simulink model "flappy_hk_disturbed_position_hover"  (R2024a)
settings: Solver=ode15s  StartTime=0.0  StopTime=5  MaxStep=0.0001  RelTol=1e-3
undefined symbols (not defined in the file): flappy_sil_position_controller, flappy_sil_sensor_model, flappy_sil_virtual_actuator, flappy_sil_wing_kinematics, flappy_sil_wing_loads, X, Y, Z
libraries: sm_lib x66, nesl_utility x36
(part 1 of 2)
settings Model: Creator=10049  LastModifiedBy=10049
settings DataIOCC: SaveFormat=StructureWithTime

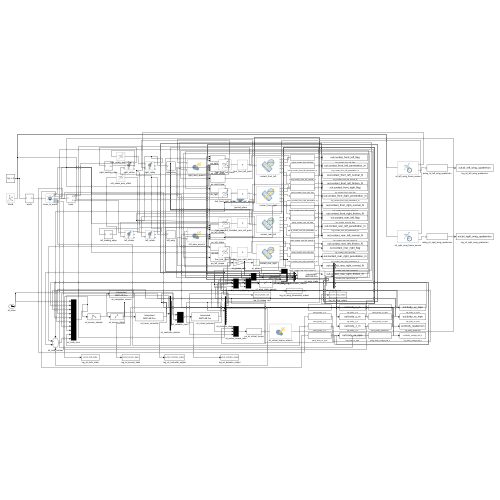
[thumbnail: Simulink's stored preview of the top-level diagram]
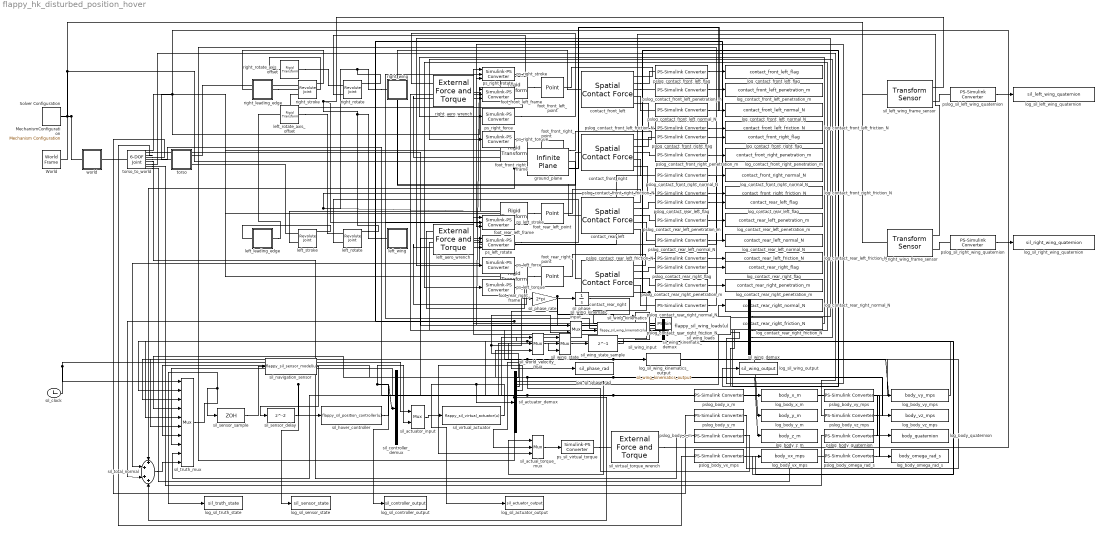
== system flappy_hk_disturbed_position_hover ==
  MechanismConfiguration : sm_lib/Utilities/Mechanism Configuration  UniformGravity=Constant  GravityVector=[0 0 -9.80665]  GravityVectorUnits=m/s^2  LinearizationDelta=0.001  JointModeTransitionNonlinearIterations=2
  Solver Configuration : nesl_utility/Solver Configuration  PhysicalDomain=network_engine_domain  SubClassName=solver  LeftPortType=input  RightPortType=generic  Tones=[]  Harmonics=[]  SimulateNoise=off  Profile=off  UseLocalSampling=off  EnableSwitchedLinearOptims=on  FrequencyDomain=off  UseCCode=off  RelTol=0.001  AbsTol=0.001  MinStep=1e-09  ToWorkspace=off  RevertToSquareIcSolve=off  NumHomotopyIterations=100  PhasorMode=off  PhasorModeNumHarmonics=1  ConsistencySolver=NEWTON_XTOL_AFTER_FTOL  IndexReductionMethod=DerivativeReplacement  DoDC=off  ResidualTolerance=1e-09  ConsistencyTolSource=GLOBAL  ConsistencyAbsTol=0.001  ConsistencyRelTol=0.001  ConsistencyTolFactor=0.001  UseLocalSolver=off  LocalSolverChoice=NE_BACKWARD_EULER_ADVANCER  ResolveIndetEquations=on  FunctionEvalNumThread=1  LocalSolverSampleTime=0.001  DoFixedCost=off  MaxNonlinIter=3  MaxModeIter=2  ComputeImpulses=off  ImpulseIterations=2  LinearAlgebra=auto  LinearAlgebraNumThread=0  EquationFormulation=NE_TIME_EF  DelaysMemoryBudget=1024  AutomaticFiltering=on  FilteringTimeConstant=0.001  PartitionStorageMethod=AS_NEEDED  PartitionMemoryBudget=1024  PartitionMethod=ROBUST  MultibodyUseLocalSolver=off  MultibodyLocalSolverChoice=ODE1  MultibodyLocalSolverSampleTime=0.001
  World : sm_lib/Frames and Transforms/World Frame
  contact_front_left : sm_lib/Forces and Torques/Spatial Contact Force  NormalForceType=SmoothSpringDamper  NormalStiffness=996.3556  NormalStiffnessUnits=N/m  NormalDamping=9.9602  NormalDampingUnits=N/(m/s)  NormalTransitionRegionWidth=0.0001  NormalTransitionRegionWidthUnits=m  FrictionType=SmoothStickSlip  CoefficientOfStaticFriction=0.6  CoefficientOfDynamicFriction=0.5  FrictionalCriticalVelocity=0.01  FrictionalCriticalVelocityUnits=m/s  SenseContactSignal=on  SensePenetrationDepth=on  SenseSeparationDistance=off  SenseNormalForceMagnitude=on  SenseFrictionalForceMagnitude=on  SenseNormalVelocity=off  SenseTangentialVelocity=off  SenseContactBaseRotation=off  SenseContactBaseTranslation=off  SenseContactFollowerRotation=off  SenseContactFollowerTranslation=off  ZeroCrossDetectContactStartAndEnd=on
  contact_front_right : sm_lib/Forces and Torques/Spatial Contact Force  NormalForceType=SmoothSpringDamper  NormalStiffness=996.3556  NormalStiffnessUnits=N/m  NormalDamping=9.9602  NormalDampingUnits=N/(m/s)  NormalTransitionRegionWidth=0.0001  NormalTransitionRegionWidthUnits=m  FrictionType=SmoothStickSlip  CoefficientOfStaticFriction=0.6  CoefficientOfDynamicFriction=0.5  FrictionalCriticalVelocity=0.01  FrictionalCriticalVelocityUnits=m/s  SenseContactSignal=on  SensePenetrationDepth=on  SenseSeparationDistance=off  SenseNormalForceMagnitude=on  SenseFrictionalForceMagnitude=on  SenseNormalVelocity=off  SenseTangentialVelocity=off  SenseContactBaseRotation=off  SenseContactBaseTranslation=off  SenseContactFollowerRotation=off  SenseContactFollowerTranslation=off  ZeroCrossDetectContactStartAndEnd=on
  contact_rear_left : sm_lib/Forces and Torques/Spatial Contact Force  NormalForceType=SmoothSpringDamper  NormalStiffness=996.3556  NormalStiffnessUnits=N/m  NormalDamping=9.9602  NormalDampingUnits=N/(m/s)  NormalTransitionRegionWidth=0.0001  NormalTransitionRegionWidthUnits=m  FrictionType=SmoothStickSlip  CoefficientOfStaticFriction=0.6  CoefficientOfDynamicFriction=0.5  FrictionalCriticalVelocity=0.01  FrictionalCriticalVelocityUnits=m/s  SenseContactSignal=on  SensePenetrationDepth=on  SenseSeparationDistance=off  SenseNormalForceMagnitude=on  SenseFrictionalForceMagnitude=on  SenseNormalVelocity=off  SenseTangentialVelocity=off  SenseContactBaseRotation=off  SenseContactBaseTranslation=off  SenseContactFollowerRotation=off  SenseContactFollowerTranslation=off  ZeroCrossDetectContactStartAndEnd=on
  contact_rear_right : sm_lib/Forces and Torques/Spatial Contact Force  NormalForceType=SmoothSpringDamper  NormalStiffness=996.3556  NormalStiffnessUnits=N/m  NormalDamping=9.9602  NormalDampingUnits=N/(m/s)  NormalTransitionRegionWidth=0.0001  NormalTransitionRegionWidthUnits=m  FrictionType=SmoothStickSlip  CoefficientOfStaticFriction=0.6  CoefficientOfDynamicFriction=0.5  FrictionalCriticalVelocity=0.01  FrictionalCriticalVelocityUnits=m/s  SenseContactSignal=on  SensePenetrationDepth=on  SenseSeparationDistance=off  SenseNormalForceMagnitude=on  SenseFrictionalForceMagnitude=on  SenseNormalVelocity=off  SenseTangentialVelocity=off  SenseContactBaseRotation=off  SenseContactBaseTranslation=off  SenseContactFollowerRotation=off  SenseContactFollowerTranslation=off  ZeroCrossDetectContactStartAndEnd=on
  foot_front_left_frame : sm_lib/Frames and Transforms/Rigid Transform  RotationMethod=None  FollAlignAxisA=+X  BaseAlignAxisA=+Y  FollAlignAxisB=+Y  BaseAlignAxisB=+Z  RotationStandardAxis=+Z  RotationAngle=0  RotationAngleUnits=deg  RotationArbitraryAxis=[0 0 1]  RotationSequenceAxes=FollowerAxes  RotationSequence=XYX  RotationSequenceAngles=[0 0 0]  RotationSequenceAnglesUnits=deg  RotationMatrix=[1 0 0;0 1 0;0 0 1]  Quaternion=[1 0 0 0]  TranslationMethod=Cartesian  TranslationCartesianOffset=[-0.056123561 -0.056123561 -0.0610087]  TranslationCartesianOffsetUnits=m  TranslationStandardAxis=+Z  TranslationStandardOffset=0  TranslationStandardOffsetUnits=m  TranslationROffset=0  TranslationROffsetUnits=m  TranslationThetaOffset=0  TranslationThetaOffsetUnits=deg  TranslationZOffset=0  TranslationZOffsetUnits=m
  foot_front_left_point : sm_lib/Curves and Surfaces/Point  GraphicType=Marker  MarkerShape=Sphere  MarkerSize=10  GraphicVisPropType=SimpleVisualProperties  GraphicDiffuseColor=[0.5 0.5 0.5]  GraphicOpacity=1  GraphicSpecularColor=[0.5 0.5 0.5 1.0]  GraphicAmbientColor=[0.15 0.15 0.15 1.0]  GraphicEmissiveColor=[0.0 0.0 0.0 1.0]  GraphicShininess=75
  foot_front_right_frame : sm_lib/Frames and Transforms/Rigid Transform  RotationMethod=None  FollAlignAxisA=+X  BaseAlignAxisA=+Y  FollAlignAxisB=+Y  BaseAlignAxisB=+Z  RotationStandardAxis=+Z  RotationAngle=0  RotationAngleUnits=deg  RotationArbitraryAxis=[0 0 1]  RotationSequenceAxes=FollowerAxes  RotationSequence=XYX  RotationSequenceAngles=[0 0 0]  RotationSequenceAnglesUnits=deg  RotationMatrix=[1 0 0;0 1 0;0 0 1]  Quaternion=[1 0 0 0]  TranslationMethod=Cartesian  TranslationCartesianOffset=[-0.056123561 0.056123557 -0.0610087]  TranslationCartesianOffsetUnits=m  TranslationStandardAxis=+Z  TranslationStandardOffset=0  TranslationStandardOffsetUnits=m  TranslationROffset=0  TranslationROffsetUnits=m  TranslationThetaOffset=0  TranslationThetaOffsetUnits=deg  TranslationZOffset=0  TranslationZOffsetUnits=m
  foot_front_right_point : sm_lib/Curves and Surfaces/Point  GraphicType=Marker  MarkerShape=Sphere  MarkerSize=10  GraphicVisPropType=SimpleVisualProperties  GraphicDiffuseColor=[0.5 0.5 0.5]  GraphicOpacity=1  GraphicSpecularColor=[0.5 0.5 0.5 1.0]  GraphicAmbientColor=[0.15 0.15 0.15 1.0]  GraphicEmissiveColor=[0.0 0.0 0.0 1.0]  GraphicShininess=75
  foot_rear_left_frame : sm_lib/Frames and Transforms/Rigid Transform  RotationMethod=None  FollAlignAxisA=+X  BaseAlignAxisA=+Y  FollAlignAxisB=+Y  BaseAlignAxisB=+Z  RotationStandardAxis=+Z  RotationAngle=0  RotationAngleUnits=deg  RotationArbitraryAxis=[0 0 1]  RotationSequenceAxes=FollowerAxes  RotationSequence=XYX  RotationSequenceAngles=[0 0 0]  RotationSequenceAnglesUnits=deg  RotationMatrix=[1 0 0;0 1 0;0 0 1]  Quaternion=[1 0 0 0]  TranslationMethod=Cartesian  TranslationCartesianOffset=[0.056357642 -0.056357654 -0.0610087]  TranslationCartesianOffsetUnits=m  TranslationStandardAxis=+Z  TranslationStandardOffset=0  TranslationStandardOffsetUnits=m  TranslationROffset=0  TranslationROffsetUnits=m  TranslationThetaOffset=0  TranslationThetaOffsetUnits=deg  TranslationZOffset=0  TranslationZOffsetUnits=m
  foot_rear_left_point : sm_lib/Curves and Surfaces/Point  GraphicType=Marker  MarkerShape=Sphere  MarkerSize=10  GraphicVisPropType=SimpleVisualProperties  GraphicDiffuseColor=[0.5 0.5 0.5]  GraphicOpacity=1  GraphicSpecularColor=[0.5 0.5 0.5 1.0]  GraphicAmbientColor=[0.15 0.15 0.15 1.0]  GraphicEmissiveColor=[0.0 0.0 0.0 1.0]  GraphicShininess=75
  foot_rear_right_frame : sm_lib/Frames and Transforms/Rigid Transform  RotationMethod=None  FollAlignAxisA=+X  BaseAlignAxisA=+Y  FollAlignAxisB=+Y  BaseAlignAxisB=+Z  RotationStandardAxis=+Z  RotationAngle=0  RotationAngleUnits=deg  RotationArbitraryAxis=[0 0 1]  RotationSequenceAxes=FollowerAxes  RotationSequence=XYX  RotationSequenceAngles=[0 0 0]  RotationSequenceAnglesUnits=deg  RotationMatrix=[1 0 0;0 1 0;0 0 1]  Quaternion=[1 0 0 0]  TranslationMethod=Cartesian  TranslationCartesianOffset=[0.056357642 0.056357642 -0.0610087]  TranslationCartesianOffsetUnits=m  TranslationStandardAxis=+Z  TranslationStandardOffset=0  TranslationStandardOffsetUnits=m  TranslationROffset=0  TranslationROffsetUnits=m  TranslationThetaOffset=0  TranslationThetaOffsetUnits=deg  TranslationZOffset=0  TranslationZOffsetUnits=m
  foot_rear_right_point : sm_lib/Curves and Surfaces/Point  GraphicType=Marker  MarkerShape=Sphere  MarkerSize=10  GraphicVisPropType=SimpleVisualProperties  GraphicDiffuseColor=[0.5 0.5 0.5]  GraphicOpacity=1  GraphicSpecularColor=[0.5 0.5 0.5 1.0]  GraphicAmbientColor=[0.15 0.15 0.15 1.0]  GraphicEmissiveColor=[0.0 0.0 0.0 1.0]  GraphicShininess=75
  ground_plane : sm_lib/Curves and Surfaces/Infinite Plane  GraphicType=Rectangle  GraphicPlaneWidth=3  GraphicPlaneWidthUnits=m  GraphicPlaneHeight=3  GraphicPlaneHeightUnits=m  GraphicVisPropType=SimpleVisualProperties  GraphicDiffuseColor=[0.93 0.94 0.96]  GraphicOpacity=0.98  GraphicSpecularColor=[0.06 0.06 0.07 1]  GraphicAmbientColor=[0.2 0.2 0.2 1]  GraphicEmissiveColor=[0 0 0 1]  GraphicShininess=4
  left_aero_wrench : sm_lib/Forces and Torques/External Force and Torque  EnableForceX=off  EnableForceY=off  EnableForceZ=off  EnableForce=on  ForceResolutionFrame=World  EnableTorqueX=off  EnableTorqueY=off  EnableTorqueZ=off  EnableTorque=on  TorqueResolutionFrame=World
  left_leading_edge : Subsystem
  left_rotate : sm_lib/Joints/Revolute Joint  JointMode=Normal  CompositeWrenchDir=FollowerOnBase  CompositeWrenchFrame=BaseFrame  SenseConstraintForce=off  SenseConstraintTorque=off  SenseTotalForce=off  SenseTotalTorque=off  PositionTargetSpecify=off  PositionTargetPriority=High  PositionTargetValue=0  PositionTargetValueUnits=deg  VelocityTargetSpecify=off  VelocityTargetPriority=High  VelocityTargetValue=0  VelocityTargetValueUnits=deg/s  EquilibriumPosition=0  EquilibriumPositionUnits=deg  SpringStiffness=0  SpringStiffnessUnits=N*m/deg  DampingCoefficient=1e-9  DampingCoefficientUnits=kg*m^2/(rad*s)  LowerLimitSpecify=on  LowerLimitBound=-0.7854  LowerLimitBoundUnits=rad  LowerLimitStiffness=1e4  LowerLimitStiffnessUnits=N*m/deg  LowerLimitDamping=10  LowerLimitDampingUnits=N*m/(deg/s)  LowerLimitTransitionRegionWidth=0.1  LowerLimitTransitionRegionWidthUnits=deg  UpperLimitSpecify=on  UpperLimitBound=0.7854  UpperLimitBoundUnits=rad  UpperLimitStiffness=1e4  UpperLimitStiffnessUnits=N*m/deg  UpperLimitDamping=10  UpperLimitDampingUnits=N*m/(deg/s)  UpperLimitTransitionRegionWidth=0.1  UpperLimitTransitionRegionWidthUnits=deg  TorqueActuationMode=ComputedTorque  MotionActuationMode=InputMotion  SensePosition=on  SenseVelocity=on  SenseAcceleration=off  SenseTorqueForce=off  SenseLowerLimitTorqueForce=off  SenseUpperLimitTorqueForce=off
  left_rotate_axis_offset : sm_lib/Frames and Transforms/Rigid Transform  RotationMethod=None  FollAlignAxisA=+X  BaseAlignAxisA=+Y  FollAlignAxisB=+Y  BaseAlignAxisB=+Z  RotationStandardAxis=+Z  RotationAngle=0  RotationAngleUnits=deg  RotationArbitraryAxis=[0 0 1]  RotationSequenceAxes=FollowerAxes  RotationSequence=XYX  RotationSequenceAngles=[0 0 0]  RotationSequenceAnglesUnits=deg  RotationMatrix=[1 0 0;0 1 0;0 0 1]  Quaternion=[1 0 0 0]  TranslationMethod=Cartesian  TranslationCartesianOffset=[0 0 0]  TranslationCartesianOffsetUnits=m  TranslationStandardAxis=+Z  TranslationStandardOffset=0  TranslationStandardOffsetUnits=m  TranslationROffset=0  TranslationROffsetUnits=m  TranslationThetaOffset=0  TranslationThetaOffsetUnits=deg  TranslationZOffset=0  TranslationZOffsetUnits=m
  left_stroke : sm_lib/Joints/Revolute Joint  JointMode=Normal  CompositeWrenchDir=FollowerOnBase  CompositeWrenchFrame=BaseFrame  SenseConstraintForce=off  SenseConstraintTorque=off  SenseTotalForce=off  SenseTotalTorque=off  PositionTargetSpecify=off  PositionTargetPriority=High  PositionTargetValue=0  PositionTargetValueUnits=deg  VelocityTargetSpecify=off  VelocityTargetPriority=High  VelocityTargetValue=0  VelocityTargetValueUnits=deg/s  EquilibriumPosition=0  EquilibriumPositionUnits=deg  SpringStiffness=0.013384  SpringStiffnessUnits=N*m/deg  DampingCoefficient=8e-9  DampingCoefficientUnits=kg*m^2/(rad*s)  LowerLimitSpecify=on  LowerLimitBound=-1.63  LowerLimitBoundUnits=rad  LowerLimitStiffness=1e4  LowerLimitStiffnessUnits=N*m/deg  LowerLimitDamping=10  LowerLimitDampingUnits=N*m/(deg/s)  LowerLimitTransitionRegionWidth=0.1  LowerLimitTransitionRegionWidthUnits=deg  UpperLimitSpecify=on  UpperLimitBound=1.63  UpperLimitBoundUnits=rad  UpperLimitStiffness=1e4  UpperLimitStiffnessUnits=N*m/deg  UpperLimitDamping=10  UpperLimitDampingUnits=N*m/(deg/s)  UpperLimitTransitionRegionWidth=0.1  UpperLimitTransitionRegionWidthUnits=deg  TorqueActuationMode=ComputedTorque  MotionActuationMode=InputMotion  SensePosition=on  SenseVelocity=on  SenseAcceleration=off  SenseTorqueForce=off  SenseLowerLimitTorqueForce=off  SenseUpperLimitTorqueForce=off
  left_wing : Subsystem
  log_body_omega_rad_s : ToWorkspace  VariableName=body_omega_rad_s  SaveFormat=Structure With Time  SampleTime=-1
  log_body_quaternion : ToWorkspace  VariableName=body_quaternion  SaveFormat=Structure With Time  SampleTime=-1
  log_body_vx_mps : ToWorkspace  VariableName=body_vx_mps  SaveFormat=Structure With Time  SampleTime=-1
  log_body_vy_mps : ToWorkspace  VariableName=body_vy_mps  SaveFormat=Structure With Time  SampleTime=-1
  log_body_vz_mps : ToWorkspace  VariableName=body_vz_mps  SaveFormat=Structure With Time  SampleTime=-1
  log_body_x_m : ToWorkspace  VariableName=body_x_m  SaveFormat=Structure With Time  SampleTime=-1
  log_body_y_m : ToWorkspace  VariableName=body_y_m  SaveFormat=Structure With Time  SampleTime=-1
  log_body_z_m : ToWorkspace  VariableName=body_z_m  SaveFormat=Structure With Time  SampleTime=-1
  log_contact_front_left_flag : ToWorkspace  VariableName=contact_front_left_flag  SaveFormat=Structure With Time  SampleTime=-1
  log_contact_front_left_friction_N : ToWorkspace  VariableName=contact_front_left_friction_N  SaveFormat=Structure With Time  SampleTime=-1
  log_contact_front_left_normal_N : ToWorkspace  VariableName=contact_front_left_normal_N  SaveFormat=Structure With Time  SampleTime=-1
  log_contact_front_left_penetration_m : ToWorkspace  VariableName=contact_front_left_penetration_m  SaveFormat=Structure With Time  SampleTime=-1
  log_contact_front_right_flag : ToWorkspace  VariableName=contact_front_right_flag  SaveFormat=Structure With Time  SampleTime=-1
  log_contact_front_right_friction_N : ToWorkspace  VariableName=contact_front_right_friction_N  SaveFormat=Structure With Time  SampleTime=-1
  log_contact_front_right_normal_N : ToWorkspace  VariableName=contact_front_right_normal_N  SaveFormat=Structure With Time  SampleTime=-1
  log_contact_front_right_penetration_m : ToWorkspace  VariableName=contact_front_right_penetration_m  SaveFormat=Structure With Time  SampleTime=-1
  log_contact_rear_left_flag : ToWorkspace  VariableName=contact_rear_left_flag  SaveFormat=Structure With Time  SampleTime=-1
  log_contact_rear_left_friction_N : ToWorkspace  VariableName=contact_rear_left_friction_N  SaveFormat=Structure With Time  SampleTime=-1
  log_contact_rear_left_normal_N : ToWorkspace  VariableName=contact_rear_left_normal_N  SaveFormat=Structure With Time  SampleTime=-1
  log_contact_rear_left_penetration_m : ToWorkspace  VariableName=contact_rear_left_penetration_m  SaveFormat=Structure With Time  SampleTime=-1
  log_contact_rear_right_flag : ToWorkspace  VariableName=contact_rear_right_flag  SaveFormat=Structure With Time  SampleTime=-1
  log_contact_rear_right_friction_N : ToWorkspace  VariableName=contact_rear_right_friction_N  SaveFormat=Structure With Time  SampleTime=-1
  log_contact_rear_right_normal_N : ToWorkspace  VariableName=contact_rear_right_normal_N  SaveFormat=Structure With Time  SampleTime=-1
  log_contact_rear_right_penetration_m : ToWorkspace  VariableName=contact_rear_right_penetration_m  SaveFormat=Structure With Time  SampleTime=-1
  log_sil_actuator_output : ToWorkspace  VariableName=sil_actuator_output  SaveFormat=Structure With Time  SampleTime=-1
  log_sil_controller_output : ToWorkspace  VariableName=sil_controller_output  SaveFormat=Structure With Time  SampleTime=-1
  log_sil_left_wing_quaternion : ToWorkspace  VariableName=sil_left_wing_quaternion  SaveFormat=Structure With Time  SampleTime=-1
  log_sil_phase_rad : ToWorkspace  VariableName=sil_phase_rad  SaveFormat=Structure With Time  SampleTime=-1
  log_sil_right_wing_quaternion : ToWorkspace  VariableName=sil_right_wing_quaternion  SaveFormat=Structure With Time  SampleTime=-1
  log_sil_sensor_state : ToWorkspace  VariableName=sil_sensor_state  SaveFormat=Structure With Time  SampleTime=-1
  log_sil_truth_state : ToWorkspace  VariableName=sil_truth_state  SaveFormat=Structure With Time  SampleTime=-1
  log_sil_wing_kinematics_output : ToWorkspace  VariableName=sil_wing_kinematics_output  SaveFormat=Structure With Time  SampleTime=-1
  log_sil_wing_output : ToWorkspace  VariableName=sil_wing_output  SaveFormat=Structure With Time  SampleTime=-1
  ps_left_force : nesl_utility/Simulink-PS Converter  PhysicalDomain=network_engine_domain  SubClassName=ps_input  LeftPortType=input  RightPortType=output  PseudoPeriodic=off  Frequencies=[]  NoiseDistribution=none  NoiseParameters=[]  Unit=N  AffineConversion=off  FilteringAndDerivatives=provide  SimscapeFilterOrder=1  InputFilterTimeConstant=0.001  UdotUserProvided=0
  ps_left_rotate : nesl_utility/Simulink-PS Converter  PhysicalDomain=network_engine_domain  SubClassName=ps_input  LeftPortType=input  RightPortType=output  PseudoPeriodic=off  Frequencies=[]  NoiseDistribution=none  NoiseParameters=[]  Unit=rad  AffineConversion=off  FilteringAndDerivatives=provide  SimscapeFilterOrder=2  InputFilterTimeConstant=1e-6  UdotUserProvided=2
  ps_left_stroke : nesl_utility/Simulink-PS Converter  PhysicalDomain=network_engine_domain  SubClassName=ps_input  LeftPortType=input  RightPortType=output  PseudoPeriodic=off  Frequencies=[]  NoiseDistribution=none  NoiseParameters=[]  Unit=rad  AffineConversion=off  FilteringAndDerivatives=provide  SimscapeFilterOrder=2  InputFilterTimeConstant=1e-6  UdotUserProvided=2
  ps_left_torque : nesl_utility/Simulink-PS Converter  PhysicalDomain=network_engine_domain  SubClassName=ps_input  LeftPortType=input  RightPortType=output  PseudoPeriodic=off  Frequencies=[]  NoiseDistribution=none  NoiseParameters=[]  Unit=N*m  AffineConversion=off  FilteringAndDerivatives=provide  SimscapeFilterOrder=1  InputFilterTimeConstant=0.001  UdotUserProvided=0
  ps_right_force : nesl_utility/Simulink-PS Converter  PhysicalDomain=network_engine_domain  SubClassName=ps_input  LeftPortType=input  RightPortType=output  PseudoPeriodic=off  Frequencies=[]  NoiseDistribution=none  NoiseParameters=[]  Unit=N  AffineConversion=off  FilteringAndDerivatives=provide  SimscapeFilterOrder=1  InputFilterTimeConstant=0.001  UdotUserProvided=0
  ps_right_rotate : nesl_utility/Simulink-PS Converter  PhysicalDomain=network_engine_domain  SubClassName=ps_input  LeftPortType=input  RightPortType=output  PseudoPeriodic=off  Frequencies=[]  NoiseDistribution=none  NoiseParameters=[]  Unit=rad  AffineConversion=off  FilteringAndDerivatives=provide  SimscapeFilterOrder=2  InputFilterTimeConstant=1e-6  UdotUserProvided=2
  ps_right_stroke : nesl_utility/Simulink-PS Converter  PhysicalDomain=network_engine_domain  SubClassName=ps_input  LeftPortType=input  RightPortType=output  PseudoPeriodic=off  Frequencies=[]  NoiseDistribution=none  NoiseParameters=[]  Unit=rad  AffineConversion=off  FilteringAndDerivatives=provide  SimscapeFilterOrder=2  InputFilterTimeConstant=1e-6  UdotUserProvided=2
  ps_right_torque : nesl_utility/Simulink-PS Converter  PhysicalDomain=network_engine_domain  SubClassName=ps_input  LeftPortType=input  RightPortType=output  PseudoPeriodic=off  Frequencies=[]  NoiseDistribution=none  NoiseParameters=[]  Unit=N*m  AffineConversion=off  FilteringAndDerivatives=provide  SimscapeFilterOrder=1  InputFilterTimeConstant=0.001  UdotUserProvided=0
  ps_sil_virtual_torque : nesl_utility/Simulink-PS Converter  PhysicalDomain=network_engine_domain  SubClassName=ps_input  LeftPortType=input  RightPortType=output  PseudoPeriodic=off  Frequencies=[]  NoiseDistribution=none  NoiseParameters=[]  Unit=N*m  AffineConversion=off  FilteringAndDerivatives=provide  SimscapeFilterOrder=1  InputFilterTimeConstant=0.001  UdotUserProvided=0
  pslog_body_omega_rad_s : nesl_utility/PS-Simulink Converter  PhysicalDomain=network_engine_domain  SubClassName=ps_output  LeftPortType=input  RightPortType=output  PseudoPeriodic=off  Frequencies=[]  VectorFormat=inherit  Unit=rad/s  AffineConversion=off
  pslog_body_quaternion : nesl_utility/PS-Simulink Converter  PhysicalDomain=network_engine_domain  SubClassName=ps_output  LeftPortType=input  RightPortType=output  PseudoPeriodic=off  Frequencies=[]  VectorFormat=inherit  Unit=1  AffineConversion=off
  pslog_body_vx_mps : nesl_utility/PS-Simulink Converter  PhysicalDomain=network_engine_domain  SubClassName=ps_output  LeftPortType=input  RightPortType=output  PseudoPeriodic=off  Frequencies=[]  VectorFormat=inherit  Unit=m/s  AffineConversion=off
  pslog_body_vy_mps : nesl_utility/PS-Simulink Converter  PhysicalDomain=network_engine_domain  SubClassName=ps_output  LeftPortType=input  RightPortType=output  PseudoPeriodic=off  Frequencies=[]  VectorFormat=inherit  Unit=m/s  AffineConversion=off
  pslog_body_vz_mps : nesl_utility/PS-Simulink Converter  PhysicalDomain=network_engine_domain  SubClassName=ps_output  LeftPortType=input  RightPortType=output  PseudoPeriodic=off  Frequencies=[]  VectorFormat=inherit  Unit=m/s  AffineConversion=off
  pslog_body_x_m : nesl_utility/PS-Simulink Converter  PhysicalDomain=network_engine_domain  SubClassName=ps_output  LeftPortType=input  RightPortType=output  PseudoPeriodic=off  Frequencies=[]  VectorFormat=inherit  Unit=m  AffineConversion=off
  pslog_body_y_m : nesl_utility/PS-Simulink Converter  PhysicalDomain=network_engine_domain  SubClassName=ps_output  LeftPortType=input  RightPortType=output  PseudoPeriodic=off  Frequencies=[]  VectorFormat=inherit  Unit=m  AffineConversion=off
  pslog_body_z_m : nesl_utility/PS-Simulink Converter  PhysicalDomain=network_engine_domain  SubClassName=ps_output  LeftPortType=input  RightPortType=output  PseudoPeriodic=off  Frequencies=[]  VectorFormat=inherit  Unit=m  AffineConversion=off
  pslog_contact_front_left_flag : nesl_utility/PS-Simulink Converter  PhysicalDomain=network_engine_domain  SubClassName=ps_output  LeftPortType=input  RightPortType=output  PseudoPeriodic=off  Frequencies=[]  VectorFormat=inherit  Unit=1  AffineConversion=off
  pslog_contact_front_left_friction_N : nesl_utility/PS-Simulink Converter  PhysicalDomain=network_engine_domain  SubClassName=ps_output  LeftPortType=input  RightPortType=output  PseudoPeriodic=off  Frequencies=[]  VectorFormat=inherit  Unit=N  AffineConversion=off
  pslog_contact_front_left_normal_N : nesl_utility/PS-Simulink Converter  PhysicalDomain=network_engine_domain  SubClassName=ps_output  LeftPortType=input  RightPortType=output  PseudoPeriodic=off  Frequencies=[]  VectorFormat=inherit  Unit=N  AffineConversion=off
  pslog_contact_front_left_penetration_m : nesl_utility/PS-Simulink Converter  PhysicalDomain=network_engine_domain  SubClassName=ps_output  LeftPortType=input  RightPortType=output  PseudoPeriodic=off  Frequencies=[]  VectorFormat=inherit  Unit=m  AffineConversion=off
  pslog_contact_front_right_flag : nesl_utility/PS-Simulink Converter  PhysicalDomain=network_engine_domain  SubClassName=ps_output  LeftPortType=input  RightPortType=output  PseudoPeriodic=off  Frequencies=[]  VectorFormat=inherit  Unit=1  AffineConversion=off
  pslog_contact_front_right_friction_N : nesl_utility/PS-Simulink Converter  PhysicalDomain=network_engine_domain  SubClassName=ps_output  LeftPortType=input  RightPortType=output  PseudoPeriodic=off  Frequencies=[]  VectorFormat=inherit  Unit=N  AffineConversion=off
  pslog_contact_front_right_normal_N : nesl_utility/PS-Simulink Converter  PhysicalDomain=network_engine_domain  SubClassName=ps_output  LeftPortType=input  RightPortType=output  PseudoPeriodic=off  Frequencies=[]  VectorFormat=inherit  Unit=N  AffineConversion=off
  pslog_contact_front_right_penetration_m : nesl_utility/PS-Simulink Converter  PhysicalDomain=network_engine_domain  SubClassName=ps_output  LeftPortType=input  RightPortType=output  PseudoPeriodic=off  Frequencies=[]  VectorFormat=inherit  Unit=m  AffineConversion=off
  pslog_contact_rear_left_flag : nesl_utility/PS-Simulink Converter  PhysicalDomain=network_engine_domain  SubClassName=ps_output  LeftPortType=input  RightPortType=output  PseudoPeriodic=off  Frequencies=[]  VectorFormat=inherit  Unit=1  AffineConversion=off
  pslog_contact_rear_left_friction_N : nesl_utility/PS-Simulink Converter  PhysicalDomain=network_engine_domain  SubClassName=ps_output  LeftPortType=input  RightPortType=output  PseudoPeriodic=off  Frequencies=[]  VectorFormat=inherit  Unit=N  AffineConversion=off
  pslog_contact_rear_left_normal_N : nesl_utility/PS-Simulink Converter  PhysicalDomain=network_engine_domain  SubClassName=ps_output  LeftPortType=input  RightPortType=output  PseudoPeriodic=off  Frequencies=[]  VectorFormat=inherit  Unit=N  AffineConversion=off
  pslog_contact_rear_left_penetration_m : nesl_utility/PS-Simulink Converter  PhysicalDomain=network_engine_domain  SubClassName=ps_output  LeftPortType=input  RightPortType=output  PseudoPeriodic=off  Frequencies=[]  VectorFormat=inherit  Unit=m  AffineConversion=off
  pslog_contact_rear_right_flag : nesl_utility/PS-Simulink Converter  PhysicalDomain=network_engine_domain  SubClassName=ps_output  LeftPortType=input  RightPortType=output  PseudoPeriodic=off  Frequencies=[]  VectorFormat=inherit  Unit=1  AffineConversion=off
  pslog_contact_rear_right_friction_N : nesl_utility/PS-Simulink Converter  PhysicalDomain=network_engine_domain  SubClassName=ps_output  LeftPortType=input  RightPortType=output  PseudoPeriodic=off  Frequencies=[]  VectorFormat=inherit  Unit=N  AffineConversion=off
  pslog_contact_rear_right_normal_N : nesl_utility/PS-Simulink Converter  PhysicalDomain=network_engine_domain  SubClassName=ps_output  LeftPortType=input  RightPortType=output  PseudoPeriodic=off  Frequencies=[]  VectorFormat=inherit  Unit=N  AffineConversion=off
  pslog_contact_rear_right_penetration_m : nesl_utility/PS-Simulink Converter  PhysicalDomain=network_engine_domain  SubClassName=ps_output  LeftPortType=input  RightPortType=output  PseudoPeriodic=off  Frequencies=[]  VectorFormat=inherit  Unit=m  AffineConversion=off
  pslog_sil_left_wing_quaternion : nesl_utility/PS-Simulink Converter  PhysicalDomain=network_engine_domain  SubClassName=ps_output  LeftPortType=input  RightPortType=output  PseudoPeriodic=off  Frequencies=[]  VectorFormat=inherit  Unit=1  AffineConversion=off
  pslog_sil_right_wing_quaternion : nesl_utility/PS-Simulink Converter  PhysicalDomain=network_engine_domain  SubClassName=ps_output  LeftPortType=input  RightPortType=output  PseudoPeriodic=off  Frequencies=[]  VectorFormat=inherit  Unit=1  AffineConversion=off
  right_aero_wrench : sm_lib/Forces and Torques/External Force and Torque  EnableForceX=off  EnableForceY=off  EnableForceZ=off  EnableForce=on  ForceResolutionFrame=World  EnableTorqueX=off  EnableTorqueY=off  EnableTorqueZ=off  EnableTorque=on  TorqueResolutionFrame=World
  right_leading_edge : Subsystem
  right_rotate : sm_lib/Joints/Revolute Joint  JointMode=Normal  CompositeWrenchDir=FollowerOnBase  CompositeWrenchFrame=BaseFrame  SenseConstraintForce=off  SenseConstraintTorque=off  SenseTotalForce=off  SenseTotalTorque=off  PositionTargetSpecify=off  PositionTargetPriority=High  PositionTargetValue=0  PositionTargetValueUnits=deg  VelocityTargetSpecify=off  VelocityTargetPriority=High  VelocityTargetValue=0  VelocityTargetValueUnits=deg/s  EquilibriumPosition=0  EquilibriumPositionUnits=deg  SpringStiffness=0  SpringStiffnessUnits=N*m/deg  DampingCoefficient=1e-9  DampingCoefficientUnits=kg*m^2/(rad*s)  LowerLimitSpecify=on  LowerLimitBound=-0.7854  LowerLimitBoundUnits=rad  LowerLimitStiffness=1e4  LowerLimitStiffnessUnits=N*m/deg  LowerLimitDamping=10  LowerLimitDampingUnits=N*m/(deg/s)  LowerLimitTransitionRegionWidth=0.1  LowerLimitTransitionRegionWidthUnits=deg  UpperLimitSpecify=on  UpperLimitBound=0.7854  UpperLimitBoundUnits=rad  UpperLimitStiffness=1e4  UpperLimitStiffnessUnits=N*m/deg  UpperLimitDamping=10  UpperLimitDampingUnits=N*m/(deg/s)  UpperLimitTransitionRegionWidth=0.1  UpperLimitTransitionRegionWidthUnits=deg  TorqueActuationMode=ComputedTorque  MotionActuationMode=InputMotion  SensePosition=on  SenseVelocity=on  SenseAcceleration=off  SenseTorqueForce=off  SenseLowerLimitTorqueForce=off  SenseUpperLimitTorqueForce=off
  right_rotate_axis_offset : sm_lib/Frames and Transforms/Rigid Transform  RotationMethod=None  FollAlignAxisA=+X  BaseAlignAxisA=+Y  FollAlignAxisB=+Y  BaseAlignAxisB=+Z  RotationStandardAxis=+Z  RotationAngle=0  RotationAngleUnits=deg  RotationArbitraryAxis=[0 0 1]  RotationSequenceAxes=FollowerAxes  RotationSequence=XYX  RotationSequenceAngles=[0 0 0]  RotationSequenceAnglesUnits=deg  RotationMatrix=[1 0 0;0 1 0;0 0 1]  Quaternion=[1 0 0 0]  TranslationMethod=Cartesian  TranslationCartesianOffset=[0 0 0]  TranslationCartesianOffsetUnits=m  TranslationStandardAxis=+Z  TranslationStandardOffset=0  TranslationStandardOffsetUnits=m  TranslationROffset=0  TranslationROffsetUnits=m  TranslationThetaOffset=0  TranslationThetaOffsetUnits=deg  TranslationZOffset=0  TranslationZOffsetUnits=m
  right_stroke : sm_lib/Joints/Revolute Joint  JointMode=Normal  CompositeWrenchDir=FollowerOnBase  CompositeWrenchFrame=BaseFrame  SenseConstraintForce=off  SenseConstraintTorque=off  SenseTotalForce=off  SenseTotalTorque=off  PositionTargetSpecify=off  PositionTargetPriority=High  PositionTargetValue=0  PositionTargetValueUnits=deg  VelocityTargetSpecify=off  VelocityTargetPriority=High  VelocityTargetValue=0  VelocityTargetValueUnits=deg/s  EquilibriumPosition=0  EquilibriumPositionUnits=deg  SpringStiffness=0.013384  SpringStiffnessUnits=N*m/deg  DampingCoefficient=8e-9  DampingCoefficientUnits=kg*m^2/(rad*s)  LowerLimitSpecify=on  LowerLimitBound=-1.63  LowerLimitBoundUnits=rad  LowerLimitStiffness=1e4  LowerLimitStiffnessUnits=N*m/deg  LowerLimitDamping=10  LowerLimitDampingUnits=N*m/(deg/s)  LowerLimitTransitionRegionWidth=0.1  LowerLimitTransitionRegionWidthUnits=deg  UpperLimitSpecify=on  UpperLimitBound=1.63  UpperLimitBoundUnits=rad  UpperLimitStiffness=1e4  UpperLimitStiffnessUnits=N*m/deg  UpperLimitDamping=10  UpperLimitDampingUnits=N*m/(deg/s)  UpperLimitTransitionRegionWidth=0.1  UpperLimitTransitionRegionWidthUnits=deg  TorqueActuationMode=ComputedTorque  MotionActuationMode=InputMotion  SensePosition=on  SenseVelocity=on  SenseAcceleration=off  SenseTorqueForce=off  SenseLowerLimitTorqueForce=off  SenseUpperLimitTorqueForce=off
  right_wing : Subsystem
  sil_actual_torque_mux : Mux  Inputs=3
  sil_actuator_demux : Demux  Outputs=12
  sil_actuator_input : Mux  Inputs=2
  sil_clock : Clock
  sil_controller_demux : Demux  Outputs=24
  sil_hover_controller : MATLABFcn  MATLABFcn=flappy_sil_position_controller(u)  OutputDimensions=24  SampleTime=0.002
  sil_left_wing_frame_sensor : sm_lib/Frames and Transforms/Transform Sensor  MeasurementFrame=Base  RotationSequence=XYX  SenseAngle=off  SenseAxis=off  SenseQ=on  SenseR=off  SenseRotationSequence=off  SenseOmegaX=off  SenseOmegaY=off  SenseOmegaZ=off  SenseOmega=off  SenseQDot=off  SenseRDot=off  SenseRotationSequenceDot=off  SenseAlphaX=off  SenseAlphaY=off  SenseAlphaZ=off  SenseAlpha=off  SenseQDDot=off  SenseRDDot=off  SenseX=off  SenseY=off  SenseZ=off  SenseXYZ=off  SenseRad=off  SenseAzim=off  SenseDist=off  SenseInc=off  SenseXDot=off  SenseYDot=off  SenseZDot=off  SenseXYZDot=off  SenseRadDot=off  SenseAzimDot=off  SenseDistDot=off  SenseIncDot=off  SenseXDDot=off  SenseYDDot=off  SenseZDDot=off  SenseXYZDDot=off  SenseRadDDot=off  SenseAzimDDot=off  SenseDistDDot=off  SenseIncDDot=off
  sil_navigation_sensor : MATLABFcn  MATLABFcn=flappy_sil_sensor_model(u)  OutputDimensions=27  SampleTime=0.002
  sil_phase : Integrator
  sil_phase_rate : Gain  Gain=2*pi
  sil_right_wing_frame_sensor : sm_lib/Frames and Transforms/Transform Sensor  MeasurementFrame=Base  RotationSequence=XYX  SenseAngle=off  SenseAxis=off  SenseQ=on  SenseR=off  SenseRotationSequence=off  SenseOmegaX=off  SenseOmegaY=off  SenseOmegaZ=off  SenseOmega=off  SenseQDot=off  SenseRDot=off  SenseRotationSequenceDot=off  SenseAlphaX=off  SenseAlphaY=off  SenseAlphaZ=off  SenseAlpha=off  SenseQDDot=off  SenseRDDot=off  SenseX=off  SenseY=off  SenseZ=off  SenseXYZ=off  SenseRad=off  SenseAzim=off  SenseDist=off  SenseInc=off  SenseXDot=off  SenseYDot=off  SenseZDot=off  SenseXYZDot=off  SenseRadDot=off  SenseAzimDot=off  SenseDistDot=off  SenseIncDot=off  SenseXDDot=off  SenseYDDot=off  SenseZDDot=off  SenseXYZDDot=off  SenseRadDDot=off  SenseAzimDDot=off  SenseDistDDot=off  SenseIncDDot=off
  sil_sensor_delay : Delay  InitialCondition=zeros(27,2)  SampleTime=0.002
  sil_sensor_sample : ZeroOrderHold  SampleTime=0.002
  sil_total_normal : Sum  Inputs=++++
  sil_truth_mux : Mux  Inputs=10
  sil_virtual_actuator : MATLABFcn  MATLABFcn=flappy_sil_virtual_actuator(u)  OutputDimensions=12  SampleTime=0.002
  sil_virtual_torque_wrench : sm_lib/Forces and Torques/External Force and Torque  EnableForceX=off  EnableForceY=off  EnableForceZ=off  EnableForce=off  ForceResolutionFrame=AttachedFrame  EnableTorqueX=off  EnableTorqueY=off  EnableTorqueZ=off  EnableTorque=on  TorqueResolutionFrame=AttachedFrame
  sil_wing_demux : Demux  Outputs=[1 1 3 3 3 3 6 8]
  sil_wing_input : Mux  Inputs=3
  sil_wing_kinematic_demux : Demux  Outputs=6
  sil_wing_kinematic_input : Mux  Inputs=2
  sil_wing_kinematics : MATLABFcn  MATLABFcn=flappy_sil_wing_kinematics(u)  OutputDimensions=6  SampleTime=0.0001
  sil_wing_loads : MATLABFcn  MATLABFcn=flappy_sil_wing_loads(u)  OutputDimensions=28  SampleTime=0.001
  sil_wing_state : Mux  Inputs=3
  sil_wing_state_sample : Delay  DelayLength=1  InitialCondition=zeros(10,1)  SampleTime=0.001
  sil_world_velocity_mux : Mux  Inputs=3
  torso : Subsystem
  torso_to_world : sm_lib/Joints/6-DOF Joint  JointMode=Normal  CompositeWrenchDir=FollowerOnBase  CompositeWrenchFrame=BaseFrame  SenseConstraintForce=off  SenseConstraintTorque=off  SenseTotalForce=off  SenseTotalTorque=off  PxPositionTargetSpecify=on  PxPositionTargetPriority=High  PxPositionTargetValue=0  PxPositionTargetValueUnits=m  PxVelocityTargetSpecify=off  PxVelocityTargetPriority=High  PxVelocityTargetValue=0  PxVelocityTargetValueUnits=m/s  PxEquilibriumPosition=0  PxEquilibriumPositionUnits=m  PxSpringStiffness=0  PxSpringStiffnessUnits=N/m  PxDampingCoefficient=0  PxDampingCoefficientUnits=N/(m/s)  PxLowerLimitSpecify=off  PxLowerLimitBound=-1  PxLowerLimitBoundUnits=m  PxLowerLimitStiffness=1e6  PxLowerLimitStiffnessUnits=N/m  PxLowerLimitDamping=1e3  PxLowerLimitDampingUnits=N/(m/s)  PxLowerLimitTransitionRegionWidth=1e-4  PxLowerLimitTransitionRegionWidthUnits=m  PxUpperLimitSpecify=off  PxUpperLimitBound=1  PxUpperLimitBoundUnits=m  PxUpperLimitStiffness=1e6  PxUpperLimitStiffnessUnits=N/m  PxUpperLimitDamping=1e3  PxUpperLimitDampingUnits=N/(m/s)  PxUpperLimitTransitionRegionWidth=1e-4  PxUpperLimitTransitionRegionWidthUnits=m  PxTorqueActuationMode=NoTorque  PxMotionActuationMode=ComputedMotion  PxSensePosition=on  PxSenseVelocity=on  PxSenseAcceleration=off  PxSenseTorqueForce=off  PxSenseLowerLimitTorqueForce=off  PxSenseUpperLimitTorqueForce=off  PyPositionTargetSpecify=on  PyPositionTargetPriority=High  PyPositionTargetValue=0  PyPositionTargetValueUnits=m  PyVelocityTargetSpecify=off  PyVelocityTargetPriority=High  PyVelocityTargetValue=0  PyVelocityTargetValueUnits=m/s  PyEquilibriumPosition=0  PyEquilibriumPositionUnits=m  PySpringStiffness=0  PySpringStiffnessUnits=N/m  PyDampingCoefficient=0  PyDampingCoefficientUnits=N/(m/s)  PyLowerLimitSpecify=off  PyLowerLimitBound=-1  PyLowerLimitBoundUnits=m  PyLowerLimitStiffness=1e6  PyLowerLimitStiffnessUnits=N/m  PyLowerLimitDamping=1e3  PyLowerLimitDampingUnits=N/(m/s)  PyLowerLimitTransitionRegionWidth=1e-4  PyLowerLimitTransitionRegionWidthUnits=m  PyUpperLimitSpecify=off  PyUpperLimitBound=1  PyUpperLimitBoundUnits=m  PyUpperLimitStiffness=1e6  PyUpperLimitStiffnessUnits=N/m  PyUpperLimitDamping=1e3  PyUpperLimitDampingUnits=N/(m/s)  PyUpperLimitTransitionRegionWidth=1e-4  PyUpperLimitTransitionRegionWidthUnits=m  PyTorqueActuationMode=NoTorque  PyMotionActuationMode=ComputedMotion  PySensePosition=on  PySenseVelocity=on  PySenseAcceleration=off  PySenseTorqueForce=off  PySenseLowerLimitTorqueForce=off  PySenseUpperLimitTorqueForce=off  PzPositionTargetSpecify=on  PzPositionTargetPriority=High  PzPositionTargetValue=0.0605087  PzPositionTargetValueUnits=m  PzVelocityTargetSpecify=off  PzVelocityTargetPriority=High  PzVelocityTargetValue=0  PzVelocityTargetValueUnits=m/s  PzEquilibriumPosition=0  PzEquilibriumPositionUnits=m  PzSpringStiffness=0  PzSpringStiffnessUnits=N/m  PzDampingCoefficient=0  PzDampingCoefficientUnits=N/(m/s)  PzLowerLimitSpecify=off  PzLowerLimitBound=-1  PzLowerLimitBoundUnits=m  PzLowerLimitStiffness=1e6  PzLowerLimitStiffnessUnits=N/m  PzLowerLimitDamping=1e3  PzLowerLimitDampingUnits=N/(m/s)  PzLowerLimitTransitionRegionWidth=1e-4  PzLowerLimitTransitionRegionWidthUnits=m  PzUpperLimitSpecify=off  PzUpperLimitBound=1  PzUpperLimitBoundUnits=m  PzUpperLimitStiffness=1e6  PzUpperLimitStiffnessUnits=N/m  PzUpperLimitDamping=1e3  PzUpperLimitDampingUnits=N/(m/s)  PzUpperLimitTransitionRegionWidth=1e-4  PzUpperLimitTransitionRegionWidthUnits=m  PzTorqueActuationMode=NoTorque  PzMotionActuationMode=ComputedMotion  PzSensePosition=on  PzSenseVelocity=on  PzSenseAcceleration=off  PzSenseTorqueForce=off  PzSenseLowerLimitTorqueForce=off  PzSenseUpperLimitTorqueForce=off  SphPositionTargetSpecify=off  SphPositionTargetPriority=High  SphPositionTargetRotationMethod=None  SphPositionTargetFollAlignAxisA=+X  SphPositionTargetBaseAlignAxisA=+Y  SphPositionTargetFollAlignAxisB=+Y  SphPositionTargetBaseAlignAxisB=+Z  SphPositionTargetRotationStandardAxis=+Z  SphPositionTargetRotationAngle=0  SphPositionTargetRotationAngleUnits=deg  SphPositionTargetRotationArbitraryAxis=[0 0 1]  SphPositionTargetRotationSequenceAxes=FollowerAxes  SphPositionTargetRotationSequence=XYX  SphPositionTargetRotationSequenceAngles=[0 0 0]  SphPositionTargetRotationSequenceAnglesUnits=deg  SphPositionTargetRotationMatrix=[1 0 0;0 1 0;0 0 1]  SphPositionTargetQuaternion=[1 0 0 0]  SphVelocityTargetSpecify=off  SphVelocityTargetPriority=High  SphVelocityTargetValue=[0 0 0]  SphVelocityTargetValueUnits=deg/s  SphVelocityTargetInFollowerFrame=on  SphEqPosRotationMethod=None  SphEqPosFollAlignAxisA=+X  SphEqPosBaseAlignAxisA=+Y  SphEqPosFollAlignAxisB=+Y  SphEqPosBaseAlignAxisB=+Z  SphEqPosRotationStandardAxis=+Z  SphEqPosRotationAngle=0  SphEqPosRotationAngleUnits=deg  SphEqPosRotationArbitraryAxis=[0 0 1]  SphEqPosRotationSequenceAxes=FollowerAxes  SphEqPosRotationSequence=XYX  SphEqPosRotationSequenceAngles=[0 0 0]  SphEqPosRotationSequenceAnglesUnits=deg  SphEqPosRotationMatrix=[1 0 0;0 1 0;0 0 1]  SphEqPosQuaternion=[1 0 0 0]  SphSpringStiffness=0  SphSpringStiffnessUnits=N*m/deg  SphDampingCoefficient=0  SphDampingCoefficientUnits=N*m/(deg/s)  SphLowerLimitSpecify=off  SphLowerLimitBound=15  SphLowerLimitBoundUnits=deg  SphLowerLimitStiffness=1e4  SphLowerLimitStiffnessUnits=N*m/deg  SphLowerLimitDamping=10  SphLowerLimitDampingUnits=N*m/(deg/s)  SphLowerLimitTransitionRegionWidth=0.1  SphLowerLimitTransitionRegionWidthUnits=deg  SphUpperLimitSpecify=off  SphUpperLimitBound=45  SphUpperLimitBoundUnits=deg  SphUpperLimitStiffness=1e4  SphUpperLimitStiffnessUnits=N*m/deg  SphUpperLimitDamping=10  SphUpperLimitDampingUnits=N*m/(deg/s)  SphUpperLimitTransitionRegionWidth=0.1  SphUpperLimitTransitionRegionWidthUnits=deg  SphTorqueActuationMode=NoTorque  SphActuateTorqueX=off  SphActuateTorqueY=off  SphActuateTorqueZ=off  SphActuateTorque=off  SphActuationFrame=BaseFrame  SphSensePosition=on  SphSenseVelocityX=off  SphSenseVelocityY=off  SphSenseVelocityZ=off  SphSenseVelocity=on  SphSenseAccelerationX=off  SphSenseAccelerationY=off  SphSenseAccelerationZ=off  SphSenseAcceleration=off  SphSenseLowerLimitTorqueMag=off  SphSenseUpperLimitTorqueMag=off  SphSensingFrame=FollowerFrame
  world : Subsystem
  wires:
  pslog_contact_front_left_flag/1 -> log_contact_front_left_flag/1
  pslog_contact_front_left_penetration_m/1 -> log_contact_front_left_penetration_m/1
  pslog_contact_front_left_normal_N/1 -> log_contact_front_left_normal_N/1, sil_total_normal/1
  pslog_contact_front_left_friction_N/1 -> log_contact_front_left_friction_N/1
  pslog_contact_front_right_flag/1 -> log_contact_front_right_flag/1
  pslog_contact_front_right_penetration_m/1 -> log_contact_front_right_penetration_m/1
  pslog_contact_front_right_normal_N/1 -> log_contact_front_right_normal_N/1, sil_total_normal/2
  pslog_contact_front_right_friction_N/1 -> log_contact_front_right_friction_N/1
  pslog_contact_rear_left_flag/1 -> log_contact_rear_left_flag/1
  pslog_contact_rear_left_penetration_m/1 -> log_contact_rear_left_penetration_m/1
  pslog_contact_rear_left_normal_N/1 -> log_contact_rear_left_normal_N/1, sil_total_normal/3
  pslog_contact_rear_left_friction_N/1 -> log_contact_rear_left_friction_N/1
  pslog_contact_rear_right_flag/1 -> log_contact_rear_right_flag/1
  pslog_contact_rear_right_penetration_m/1 -> log_contact_rear_right_penetration_m/1
  pslog_contact_rear_right_normal_N/1 -> log_contact_rear_right_normal_N/1, sil_total_normal/4
  pslog_contact_rear_right_friction_N/1 -> log_contact_rear_right_friction_N/1
  pslog_body_x_m/1 -> log_body_x_m/1, sil_truth_mux/2
  pslog_body_vx_mps/1 -> log_body_vx_mps/1, sil_truth_mux/5, sil_world_velocity_mux/1
  pslog_body_y_m/1 -> log_body_y_m/1, sil_truth_mux/3
  pslog_body_vy_mps/1 -> log_body_vy_mps/1, sil_truth_mux/6, sil_world_velocity_mux/2
  pslog_body_z_m/1 -> log_body_z_m/1, sil_truth_mux/4
  pslog_body_vz_mps/1 -> log_body_vz_mps/1, sil_truth_mux/7, sil_world_velocity_mux/3
  pslog_body_quaternion/1 -> log_body_quaternion/1, sil_truth_mux/8, sil_wing_state/1
  pslog_body_omega_rad_s/1 -> log_body_omega_rad_s/1, sil_truth_mux/9, sil_wing_state/2
  sil_clock/1 -> sil_truth_mux/1, sil_actuator_input/1
  sil_total_normal/1 -> sil_truth_mux/10
  sil_truth_mux/1 -> sil_sensor_sample/1, log_sil_truth_state/1
  sil_sensor_delay/1 -> sil_hover_controller/1, log_sil_sensor_state/1
  sil_hover_controller/1 -> sil_actuator_input/2, sil_controller_demux/1, log_sil_controller_output/1
  sil_actuator_input/1 -> sil_virtual_actuator/1
  sil_virtual_actuator/1 -> sil_actuator_demux/1, log_sil_actuator_output/1
  sil_actuator_demux/1 -> sil_phase_rate/1, sil_wing_input/2, sil_wing_kinematic_input/2
  sil_phase_rate/1 -> sil_phase/1
  sil_phase/1 -> sil_wing_input/1, sil_wing_kinematic_input/1, log_sil_phase_rad/1
  sil_wing_kinematic_input/1 -> sil_wing_kinematics/1
  sil_wing_kinematics/1 -> sil_wing_kinematic_demux/1, log_sil_wing_kinematics_output/1
  sil_world_velocity_mux/1 -> sil_wing_state/3
  sil_wing_state/1 -> sil_wing_state_sample/1
  sil_wing_state_sample/1 -> sil_wing_input/3
  sil_wing_input/1 -> sil_wing_loads/1
  sil_wing_loads/1 -> sil_wing_demux/1, log_sil_wing_output/1
  sil_wing_kinematic_demux/1 -> ps_left_stroke/1, ps_right_stroke/1
  sil_wing_kinematic_demux/3 -> ps_left_stroke/2, ps_right_stroke/2
  sil_wing_kinematic_demux/5 -> ps_left_stroke/3, ps_right_stroke/3
  sil_wing_kinematic_demux/2 -> ps_left_rotate/1, ps_right_rotate/1
  sil_wing_kinematic_demux/4 -> ps_left_rotate/2, ps_right_rotate/2
  sil_wing_kinematic_demux/6 -> ps_left_rotate/3, ps_right_rotate/3
  sil_wing_demux/3 -> ps_left_force/1
  sil_wing_demux/4 -> ps_right_force/1
  sil_wing_demux/5 -> ps_left_torque/1
  sil_wing_demux/6 -> ps_right_torque/1
  sil_actuator_demux/2 -> sil_actual_torque_mux/1
  sil_actuator_demux/3 -> sil_actual_torque_mux/2
  sil_actuator_demux/4 -> sil_actual_torque_mux/3
  sil_actual_torque_mux/1 -> ps_sil_virtual_torque/1
  pslog_sil_left_wing_quaternion/1 -> log_sil_left_wing_quaternion/1
  pslog_sil_right_wing_quaternion/1 -> log_sil_right_wing_quaternion/1
  sil_sensor_sample/1 -> sil_navigation_sensor/1
  sil_navigation_sensor/1 -> sil_sensor_delay/1
  connections:
  left_leading_edge/LConn1 -- left_stroke/RConn1
  MechanismConfiguration/RConn1 -- Solver Configuration/RConn1 -- world/LConn1 -- ground_plane/LConn1 -- sil_left_wing_frame_sensor/LConn1 -- World/RConn1 -- sil_right_wing_frame_sensor/LConn1
  left_wing/LConn1 -- left_rotate/RConn1 -- left_aero_wrench/RConn1 -- sil_left_wing_frame_sensor/RConn1
  right_leading_edge/LConn1 -- right_stroke/RConn1
  right_wing/LConn1 -- right_rotate/RConn1 -- right_aero_wrench/RConn1 -- sil_right_wing_frame_sensor/RConn1
  torso_to_world/RConn1 -- torso/LConn1 -- foot_front_left_frame/LConn1 -- foot_front_right_frame/LConn1 -- foot_rear_left_frame/LConn1 -- foot_rear_right_frame/LConn1 -- sil_virtual_torque_wrench/RConn1
  left_stroke/LConn1 -- torso/RConn2
  right_stroke/LConn1 -- torso/RConn1
  torso_to_world/LConn1 -- world/RConn1
  left_leading_edge/RConn1 -- left_rotate_axis_offset/LConn1
  left_rotate_axis_offset/RConn1 -- left_rotate/LConn1
  right_leading_edge/RConn1 -- right_rotate_axis_offset/LConn1
  right_rotate_axis_offset/RConn1 -- right_rotate/LConn1
  ps_left_stroke/RConn1 -- left_stroke/LConn2
  ps_left_rotate/RConn1 -- left_rotate/LConn2
  ps_right_stroke/RConn1 -- right_stroke/LConn2
  ps_right_rotate/RConn1 -- right_rotate/LConn2
  ps_left_force/RConn1 -- left_aero_wrench/LConn1
  ps_left_torque/RConn1 -- left_aero_wrench/LConn2
  ps_right_force/RConn1 -- right_aero_wrench/LConn1
  ps_right_torque/RConn1 -- right_aero_wrench/LConn2
  foot_front_left_frame/RConn1 -- foot_front_left_point/LConn1
  contact_front_left/LConn1 -- ground_plane/RConn1 -- contact_front_right/LConn1 -- contact_rear_left/LConn1 -- contact_rear_right/LConn1
  foot_front_left_point/RConn1 -- contact_front_left/RConn1
  contact_front_left/RConn2 -- pslog_contact_front_left_flag/LConn1
  contact_front_left/RConn3 -- pslog_contact_front_left_penetration_m/LConn1
  contact_front_left/RConn4 -- pslog_contact_front_left_normal_N/LConn1
  contact_front_left/RConn5 -- pslog_contact_front_left_friction_N/LConn1
  foot_front_right_frame/RConn1 -- foot_front_right_point/LConn1
  foot_front_right_point/RConn1 -- contact_front_right/RConn1
  contact_front_right/RConn2 -- pslog_contact_front_right_flag/LConn1
  contact_front_right/RConn3 -- pslog_contact_front_right_penetration_m/LConn1
  contact_front_right/RConn4 -- pslog_contact_front_right_normal_N/LConn1
  contact_front_right/RConn5 -- pslog_contact_front_right_friction_N/LConn1
  foot_rear_left_frame/RConn1 -- foot_rear_left_point/LConn1
  foot_rear_left_point/RConn1 -- contact_rear_left/RConn1
  contact_rear_left/RConn2 -- pslog_contact_rear_left_flag/LConn1
  contact_rear_left/RConn3 -- pslog_contact_rear_left_penetration_m/LConn1
  contact_rear_left/RConn4 -- pslog_contact_rear_left_normal_N/LConn1
  contact_rear_left/RConn5 -- pslog_contact_rear_left_friction_N/LConn1
  foot_rear_right_frame/RConn1 -- foot_rear_right_point/LConn1
  foot_rear_right_point/RConn1 -- contact_rear_right/RConn1
  contact_rear_right/RConn2 -- pslog_contact_rear_right_flag/LConn1
  contact_rear_right/RConn3 -- pslog_contact_rear_right_penetration_m/LConn1
  contact_rear_right/RConn4 -- pslog_contact_rear_right_normal_N/LConn1
  contact_rear_right/RConn5 -- pslog_contact_rear_right_friction_N/LConn1
  torso_to_world/RConn2 -- pslog_body_x_m/LConn1
  torso_to_world/RConn3 -- pslog_body_vx_mps/LConn1
  torso_to_world/RConn4 -- pslog_body_y_m/LConn1
  torso_to_world/RConn5 -- pslog_body_vy_mps/LConn1
  torso_to_world/RConn6 -- pslog_body_z_m/LConn1
  torso_to_world/RConn7 -- pslog_body_vz_mps/LConn1
  torso_to_world/RConn8 -- pslog_body_quaternion/LConn1
  torso_to_world/RConn9 -- pslog_body_omega_rad_s/LConn1
  ps_sil_virtual_torque/RConn1 -- sil_virtual_torque_wrench/LConn1
  sil_left_wing_frame_sensor/RConn2 -- pslog_sil_left_wing_quaternion/LConn1
  sil_right_wing_frame_sensor/RConn2 -- pslog_sil_right_wing_quaternion/LConn1
